simulink model "mars_rover_terrain"  (R2025a)
settings: Solver=daessc  StartTime=0.0  StopTime=130*10  FixedStep=1e-10  MaxStep=1e-1  RelTol=1e-3  AbsTol=1e-3  EnableMultiTasking=on
undefined symbols (not defined in the file): arm_q0, Control, eeConfig, L1, L2, L3, LS1, LS3, R1, R2, R3, Rover, rover_path, RS1, RS3, X, Y, Z
libraries: sm_lib x137, nesl_utility x109, fl_lib x85, sdl_lib x20, ee_lib x10, mars_rover_lib x8, simulink x4, slpidlib x3, batteryecm_lib x2, robotcorelib x1, robotalgslib x1
(part 1 of 10)
Description:
  | Mars Rover on Uneven Terrain
  | Copyright 2022-2025 The MathWorks, Inc.
settings Model: VariantFading=off  Creator=The MathWorks, Inc.  LastModifiedBy=smiller
settings SolverCC: AutoScaleAbsTol=off  MaxConsecutiveZCs=500  AlgebraicLoopSolver=TrustRegion  MinimalZcImpactIntegration=on
settings DataIOCC: MaxDataPoints=10000  SaveFormat=Array  ReturnWorkspaceOutputs=off  SignalLoggingName=logsout_mars_rover_terrain
settings OptimizationCC: ReuseModelBlockBuffer=off  LifeSpan=inf
settings DebuggingCC: UnconnectedInputMsg=warning  UnconnectedOutputMsg=warning  UnconnectedLineMsg=warning  AllowSymbolicDim=off  SFUnexpectedBacktrackingDiag=warning  SFNoUnconditionalDefaultTransitionDiag=warning  SFExecutionAtInitializationDiag=none  ArithmeticOperatorsInVariantConditions=warning
settings ModelReferenceCC: EnableRefExpFcnMdlSchedulingChecks=on
settings SFSimCC: SimUseLocalCustomCode=off  CustomCodeUndefinedFunction=UseInterfaceOnly
settings RTWCC: RTWUseLocalCustomCode=off  GPUComputeCapability=3.5  DLArmComputeVersion=19.05
settings CodeAppCC: StateflowObjectComments=on
settings GRTTargetCC: TargetLangStandard=C89/C90 (ANSI)
settings ConfigComp: CovMetricSettings=dw  CovSaveCumulativeToWorkspaceVar=on  CovSaveSingleToWorkspaceVar=on  CovExternalEMLEnable=off  CovSFcnEnable=off
settings SimscapeCC: SimscapeLogType=all  SimscapeLogSimulationStatistics=on  SimscapeLogName=simlog_mars_rover_terrain  SimscapeLogLimitData=off  SimscapeLogDataHistory=10000.0  SimscapeOperatingPoint=sm_mars_rover_op
settings DiagnosticsConfigSet: SimMechanicsConflictingReferenceFrames=none
settings ExplorerConfigSet: InternalSimMechanicsExplorerSettings="<ExplorerConfiguration><canonicalview>default</canonicalview><AnimationSetting><BasePlaybackSpeed>1.0</BasePlaybackSpeed><PlaybackSpeedFactor>16.0</PlaybackSpeedFactor></AnimationSetting><TilePanel><TileInfo><Tiles Columns=\"1\" Count=\"1\" Rows=\"1\"><Column Weight=\"1\"/><Row Weight=\"1\"/><Tile Height=\"1\" Width=\"1\" X=\"0\" Y=\"0\"/></Tiles></TileInfo><SceneInfo><SceneViewer><BGColor><R>0.819607853889465332</R><G>0.709803938865661621</G><B>0.662745118141174316</B></BGColor><Camera><DoPerspective>on</DoPerspective><Position><X>58.577415517520329</X><Y>32.9050911370938053</Y><Z>3.55732420536288174</Z></Position><Center><X>58.5375750727138282</X><Y>33.8739693483205073</Y><Z>3.31301343857646291</Z></Center><Up><X>0</X><Y>0</Y><Z>1</Z></Up><ViewLimDist>1</ViewLimDist><YLim>0.466307658154998583</YLim><XLim>1.07946358434775913</XLim></Camera></SceneViewer></SceneInfo></TilePanel><MechEditorPanel><Cameras><Camera><Id>Camera7</Id><Value><Name>Chassis_Rear</Name><NativeCamera><PositionTrackingFeature>Rover.Chassis.Chassis.Camera_Frames.Reference_Chassis_Camera_Rear.R</PositionTrackingFeature><CenterTrackingFeature>Rover.Chassis.Chassis.Camera_Frames.Reference_Chassis_Camera_Rear.R</CenterTrackingFeature><UpVectorTrackingFeature>Rover.World_Frame.W</UpVectorTrackingFeature><CenterTrackingOrigin>off</CenterTrackingOrigin><CenterTrackingDirection>-Y</CenterTrackingDirection><UpVectorTrackingDirection>+Z</UpVectorTrackingDirection></NativeCamera></Value></Camera><Camera><Id>Camera8</Id><Value><Name>Chassis_Right</Name><NativeCamera><PositionTrackingFeature>Rover.Chassis.Chassis.Camera_Frames.Reference_Chassis_Camera_Right.R</PositionTrackingFeature><CenterTrackingFeature>Rover.Chassis.Chassis.Camera_Frames.Reference_Chassis_Camera_Right.R</CenterTrackingFeature><UpVectorTrackingFeature>Rover.World_Frame.W</UpVectorTrackingFeature><CenterTrackingOrigin>off</CenterTrackingOrigin><CenterTrackingDirection>+X</CenterTrackingDirection><UpVectorTrackingDirection>+Z</UpVectorTrackingDirection></NativeCamera></Value></Camera><Camera><Id>Camera9</Id><Value><Name>Chassis_Top</Name><NativeCamera><PositionTrackingFeature>Rover.Chassis.Chassis.Camera_Frames.Reference_Chassis_Camera_Top.R</PositionTrackingFeature><CenterTrackingFeature>Rover.Chassis.Chassis.Camera_Frames.Reference_Chassis_Camera_Top.R</CenterTrackingFeature><UpVectorTrackingFeature>Rover.World_Frame.W</UpVectorTrackingFeature><CenterTrackingOrigin>off</CenterTrackingOrigin><CenterTrackingDirection>-Z</CenterTrackingDirection><UpVectorTrackingDirection>+Y</UpVectorTrackingDirection></NativeCamera></Value></Camera><Camera><Id>Camera10</Id><Value><Name>Whl_L1</Name><NativeCamera><PositionTrackingFeature>Rover.Chassis.Roll_and_Steer.Drive.Camera_Frame_L1.Reference_Cam_Whl.R</PositionTrackingFeature><CenterTrackingFeature>Rover.Chassis.Roll_and_Steer.Drive.Camera_Frame_L1.Reference_Cam_Whl.R</CenterTrackingFeature><UpVectorTrackingFeature>Rover.Chassis.Roll_and_Steer.Drive.Camera_Frame_L1.Reference_Cam_Whl.R</UpVectorTrackingFeature><CenterTrackingOrigin>off</CenterTrackingOrigin><CenterTrackingDirection>-Z</CenterTrackingDirection><UpVectorTrackingDirection>+X</UpVectorTrackingDirection></NativeCamera></Value></Camera><Camera><Id>Camera11</Id><Value><Name>Whl_R1</Name><NativeCamera><PositionTrackingFeature>Rover.Chassis.Roll_and_Steer.Drive.Camera_Frame_R1.Reference_Cam_Whl.R</PositionTrackingFeature><CenterTrackingFeature>Rover.Chassis.Roll_and_Steer.Drive.Camera_Frame_R1.Reference_Cam_Whl.R</CenterTrackingFeature><UpVectorTrackingFeature>Rover.Chassis.Roll_and_Steer.Drive.Camera_Frame_R1.Reference_Cam_Whl.R</UpVectorTrackingFeature><CenterTrackingOrigin>off</CenterTrackingOrigin><CenterTrackingDirection>+Z</CenterTrackingDirection><UpVectorTrackingDirection>-X</UpVectorTrackingDirection></NativeCamera></Value></Camera><Camera><Id>Camera12</Id><Value><Name>Whl_L2</Name><NativeCamera><PositionTrackingFeature>Rover.Chassis.Roll_and_Steer.Drive.Camera_Frame_L2.Reference_Cam_Whl.R</PositionTrackingFeature><CenterTrackingFeature>Rover.Chassis.Roll_and_Steer.Drive.Camera_Frame_L2.Reference_Cam_Whl.R</CenterTrackingFeature><UpVectorTrackingFeature>Rover.Chassis.Roll_and_Steer.Drive.Camera_Frame_L2.Reference_Cam_Whl.R</UpVectorTrackingFeature><CenterTrackingOrigin>off</CenterTrackingOrigin><CenterTrackingDirection>-Z</CenterTrackingDirection><UpVectorTrackingDirection>-Y</UpVectorTrackingDirection></NativeCamera></Value></Camera><Camera><Id>Camera13</Id><Value><Name>Whl_R2</Name><NativeCamera><PositionTrackingFeature>Rover.Chassis.Roll_and_Steer.Drive.Camera_Frame_R2.Reference_Cam_Whl.R</PositionTrackingFeature><CenterTrackingFeature>Rover.Chassis.Roll_and_Steer.Drive.Camera_Frame_R2.Reference_Cam_Whl.R</CenterTrackingFeature><UpVectorTrackingFeature>Rover.Chassis.Roll_and_Steer.Drive.Camera_Frame_R2.Reference_Cam_Whl.R</UpVectorTrackingFeature><CenterTrackingOrigin>off</CenterTrackingOrigin><CenterTrackingDirection>+Z</CenterTrackingDirection><UpVectorTrackingDirection>+Y</UpVectorTrackingDirection></NativeCamera></Value></Camera><Camera><Id>Camera14</Id><Value><Name>Whl_L3</Name><NativeCamera><PositionTrackingFeature>Rover.Chassis.Roll_and_Steer.Drive.Camera_Frame_L3.Reference_Cam_Whl.R</PositionTrackingFeature><CenterTrackingFeature>Rover.Chassis.Roll_and_Steer.Drive.Camera_Frame_L3.Reference_Cam_Whl.R</CenterTrackingFeature><UpVectorTrackingFeature>Rover.Chassis.Roll_and_Steer.Drive.Camera_Frame_L3.Reference_Cam_Whl.R</UpVectorTrackingFeature><CenterTrackingOrigin>off</CenterTrackingOrigin><CenterTrackingDirection>-Z</CenterTrackingDirection><UpVectorTrackingDirection>+X</UpVectorTrackingDirection></NativeCamera></Value></Camera><Camera><Id>Camera15</Id><Value><Name>Whl_R3</Name><NativeCamera><PositionTrackingFeature>Rover.Chassis.Roll_and_Steer.Drive.Camera_Frame_R3.Reference_Cam_Whl.R</PositionTrackingFeature><CenterTrackingFeature>Rover.Chassis.Roll_and_Steer.Drive.Camera_Frame_R3.Reference_Cam_Whl.R</CenterTrackingFeature><UpVectorTrackingFeature>Rover.Chassis.Roll_and_Steer.Drive.Camera_Frame_R3.Reference_Cam_Whl.R</UpVectorTrackingFeature><CenterTrackingOrigin>off</CenterTrackingOrigin><CenterTrackingDirection>+Z</CenterTrackingDirection><UpVectorTrackingDirection>-X</UpVectorTrackingDirection></NativeCamera></Value></Camera><Camera><Id>Camera16</Id><Value><Name>Chassis_FR</Name><NativeCamera><PositionTrackingFeature>Rover.Chassis.Chassis.Camera_Frames.Reference_Chassis_Camera_FR.R</PositionTrackingFeature><CenterTrackingFeature>Rover.Chassis.Chassis.Camera_Frames.Reference_Chassis_Camera_FR.R</CenterTrackingFeature><UpVectorTrackingFeature>Rover.World_Frame.W</UpVectorTrackingFeature><CenterTrackingOrigin>off</CenterTrackingOrigin><CenterTrackingDirection>+X</CenterTrackingDirection><UpVectorTrackingDirection>+Z</UpVectorTrackingDirection></NativeCamera></Value></Camera><Camera><Id>Camera17</Id><Value><Name>Chassis_Front</Name><NativeCamera><PositionTrackingFeature>Rover.Chassis.Chassis.Camera_Frames.Reference_Chassis_Camera_Front.R</PositionTrackingFeature><CenterTrackingFeature>Rover.Chassis.Chassis.Camera_Frames.Reference_Chassis_Camera_Front.R</CenterTrackingFeature><UpVectorTrackingFeature>Rover.World_Frame.W</UpVectorTrackingFeature><CenterTrackingOrigin>off</CenterTrackingOrigin><CenterTrackingDirection>+X</CenterTrackingDirection><UpVectorTrackingDirection>+Z</UpVectorTrackingDirection></NativeCamera></Value></Camera><Camera><Id>Camera18</Id><Value><Name>Chassis_WhlFR</Name><NativeCamera><PositionTrackingFeature>Rover.Chassis.Chassis.Camera_Frames.Reference_Chassis_Camera_WhlFR.R</PositionTrackingFeature><CenterTrackingFeature>Rover.Chassis.Chassis.Camera_Frames.Reference_Chassis_Camera_WhlFR.R</CenterTrackingFeature><UpVectorTrackingFeature>Rover.World_Frame.W</UpVectorTrackingFeature><CenterTrackingOrigin>off</CenterTrackingOrigin><CenterTrackingDirection>+X</CenterTrackingDirection><UpVectorTrackingDirection>+Z</UpVectorTrackingDirection></NativeCamera></Value></Camera><Camera><Id>Camera19</Id><Value><Name>Chassis_WhlRR</Name><NativeCamera><PositionTrackingFeature>Rover.Chassis.Chassis.Camera_Frames.Reference_Chassis_Camera_WhlRR.R</PositionTrackingFeature><CenterTrackingFeature>Rover.Chassis.Chassis.Camera_Frames.Reference_Chassis_Camera_WhlRR.R</CenterTrackingFeature><UpVectorTrackingFeature>Rover.World_Frame.W</UpVectorTrackingFeature><CenterTrackingOrigin>off</CenterTrackingOrigin><CenterTrackingDirection>+X</CenterTrackingDirection><UpVectorTrackingDirection>+Z</UpVectorTrackingDirection></NativeCamera></Value></Camera><Camera><Id>Camera20</Id><Value><Name>Chassis_Camera_Lens</Name><NativeCamera><PositionTrackingFeature>Rover.Chassis.Camera.rsm_head_1_RIGID.Reference_Camera.R</PositionTrackingFeature><CenterTrackingFeature>Rover.Chassis.Camera.rsm_head_1_RIGID.Reference_Camera.R</CenterTrackingFeature><UpVectorTrackingFeature>Rover.Chassis.Camera.rsm_head_1_RIGID.Reference_Camera.R</UpVectorTrackingFeature><CenterTrackingOrigin>off</CenterTrackingOrigin><CenterTrackingDirection>+Z</CenterTrackingDirection><UpVectorTrackingDirection>+X</UpVectorTrackingDirection></NativeCamera></Value></Camera></Cameras><GfxPanelCameraMap><MapElement CameraMLId=\"Camera8\" GfxPanelIndex=\"0\"/></GfxPanelCameraMap><VideoCreator><PlaybackSpeedRatio>1.0</PlaybackSpeedRatio><FrameRate>30</FrameRate><VideoFormat>MPEG-4</VideoFormat><FrameSize>auto</FrameSize></VideoCreator></MechEditorPanel></ExplorerConfiguration>"

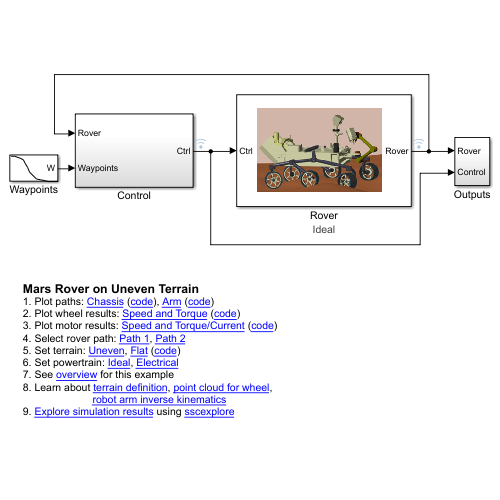
[thumbnail: Simulink's stored preview of the top-level diagram]
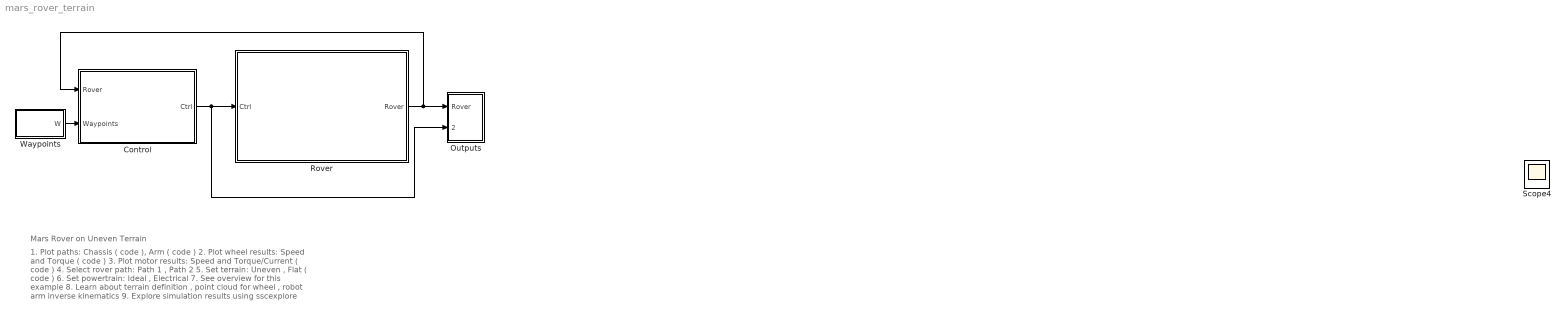
== system mars_rover_terrain ==
  note: Mars Rover on Uneven Terrain
  note: 1. Plot paths: Chassis ( code ), Arm ( code )
      | 2. Plot wheel results: Speed and Torque ( code )
      | 3. Plot motor results: Speed and Torque/Current ( code )
      | 4. Select rover path: Path 1 , Path 2
      | 5. Set terrain: Uneven , Flat ( code )
      | 6. Set powertrain: Ideal , Electrical
      | 7. See overview for this example
      | 8. Learn about terrain definition , point cloud for wheel ,
      | robot arm inverse kinematics
      | 9. Explore simulation results using sscexplore
  Control : Subsystem
  Outputs : Subsystem
  Rover : Subsystem
      mask init:
      | set_param(gcb,'AttributesFormatString',get_param([gcb '/Chassis/Powertrain'],'LabelModeActiveChoice'))
      settings: AttributesFormatString=Ideal
      mask Display: image('mars_rover_terrain_rover.png')
  Waypoints : Subsystem
      mask Display:
      | px = evalin('base','rover_path.x');
      | py = evalin('base','rover_path.y');
      | plot(px,py)
  Scope4 : Scope
      settings: ActiveDisplayYMinimum=-0.1776  ActiveDisplayYMaximum=0.10656  DataLoggingVariableName=ScopeData5
  wires:
  Waypoints/1(W) -> Control/2(Waypoints)
  Control/1(Ctrl) -> Outputs/2(Control), Rover/1(Ctrl)
  Rover/1(Rover) -> Control/1(Rover), Outputs/1(Rover)

== system mars_rover_terrain/Control ==
  In Bus Element : Inport  PortName=Rover  Element=Arm
  In Bus Element1 : Inport  PortName=Rover  Element=Chassis
  In Bus Element3 : Inport  PortName=Rover  Element=Sample
  In Bus Element5 : Inport  PortName=Rover  Element=Body
  Waypoints : Inport  Port=2
  Arm Control : Subsystem
  Chassis Control : Subsystem
  Out Bus Element : Outport  PortName=Ctrl  Element=Arm
  Out Bus Element1 : Outport  PortName=Ctrl  Element=Chassis
  wires:
  Chassis Control/1(RoverAtGoal) -> Arm Control/3(RoverAtGoal)
  Arm Control/1(Ctrl) -> Out Bus Element/1
  Waypoints/1 -> Chassis Control/1(Waypoints)
  Chassis Control/2(Ctrl) -> Out Bus Element1/1
  In Bus Element/1 -> Arm Control/1(Arm)
  In Bus Element1/1 -> Chassis Control/2(Chassis)
  In Bus Element3/1 -> Arm Control/2(Sensing)
  In Bus Element5/1 -> Chassis Control/3(Body)

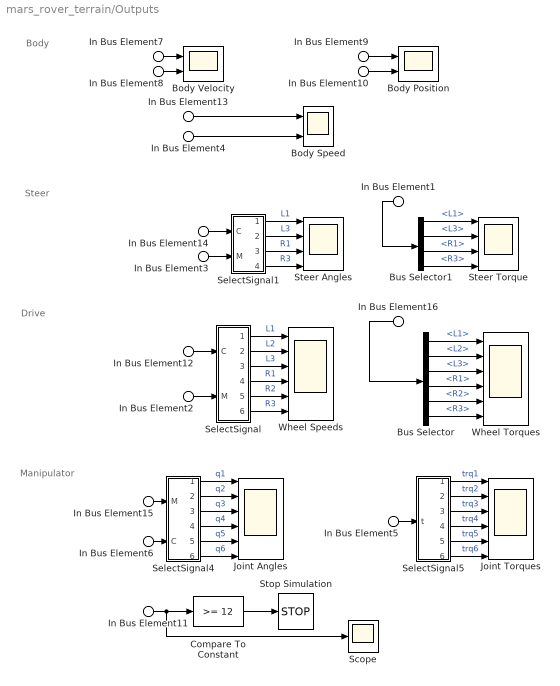
== system mars_rover_terrain/Outputs ==
  note: Body
  note: Steer
  note: Drive
  note: Manipulator
  In Bus Element2 : Inport  PortName=Rover  Element=Chassis.Wheels.Drive
  In Bus Element16 : Inport  PortName=Rover  Element=Chassis.Wheels.Drive.trq
  In Bus Element3 : Inport  PortName=Rover  Element=Chassis.Wheels.Steer
  In Bus Element15 : Inport  PortName=Rover  Element=Arm.q
  In Bus Element7 : Inport  PortName=Rover  Element=Body.vxy
  In Bus Element8 : Inport  PortName=Rover  Element=Body.wz
  In Bus Element9 : Inport  PortName=Rover  Element=Body.xyz
  In Bus Element10 : Inport  PortName=Rover  Element=Body.rpy
  In Bus Element4 : Inport  PortName=Rover  Element=Body.v
  In Bus Element1 : Inport  Port=2  PortName=Control  Element=Chassis.Steer
  In Bus Element12 : Inport  Port=2  PortName=Control  Element=Chassis.Cmd.wWhl
  In Bus Element13 : Inport  Port=2  PortName=Control  Element=Chassis.Cmd.v
  In Bus Element14 : Inport  Port=2  PortName=Control  Element=Chassis.Cmd.qSteer
  In Bus Element5 : Inport  Port=2  PortName=Control  Element=Arm.trq
  In Bus Element6 : Inport  Port=2  PortName=Control  Element=Arm.qCmd
  In Bus Element11 : Inport  Port=2  PortName=Control  Element=Arm.Mode
  Body Position : Scope  NumInputPorts=2
      settings: Title=Rover Position and Orientation  ActiveDisplayYMinimum=-4.54452  ActiveDisplayYMaximum=67.13718  YLabel=Rover XYZ Position (m)  DataLoggingVariableName=ScopeData2
  Body Speed : Scope  NumInputPorts=2
      settings: ActiveDisplayYMinimum=-0.0042  ActiveDisplayYMaximum=0.03782  DataLoggingVariableName=ScopeData7
  Body Velocity : Scope  NumInputPorts=2
      settings: Title=Rover Linear and Ang Velocities  ActiveDisplayYMinimum=-0.35082  ActiveDisplayYMaximum=0.38387  YLabel=Rover Linear Vel (m/s)
  Bus Selector : BusSelector  OutputSignals=L1,L2,L3,R1,R2,R3
  Bus Selector1 : BusSelector  OutputSignals=trq.L1,trq.L3,trq.R1,trq.R3
  Compare To Constant : simulink/Logic and Bit Operations/Compare To Constant  relop=>=  const=12  OutDataTypeStr=boolean
  Joint Angles : Scope  NumInputPorts=6
      settings: Title=Joint 1  ActiveDisplayYMinimum=-13.90292  ActiveDisplayYMaximum=99.39774  YLabel=Joint Angle (deg)  DataLoggingVariableName=ScopeData2
  Joint Torques : Scope  NumInputPorts=6
      settings: Title=Joint 1  ActiveDisplayYMinimum=-1231.55572  ActiveDisplayYMaximum=1377.74123  YLabel=Torque (N*m)
  Scope : Scope
      settings: ActiveDisplayYMinimum=-1.5  ActiveDisplayYMaximum=13.5
  SelectSignal : Subsystem
  SelectSignal1 : Subsystem
  SelectSignal4 : Subsystem
  SelectSignal5 : Subsystem
  Steer Angles : Scope  NumInputPorts=4
      settings: ActiveDisplayYMinimum=-23.51402  ActiveDisplayYMaximum=36.5986  YLabel=Steer Angle (Deg)  DataLoggingVariableName=ScopeData3
  Steer Torque : Scope  NumInputPorts=4
      settings: ActiveDisplayYMinimum=-139.38584  ActiveDisplayYMaximum=135.19843  YLabel=Torque (N*m)  DataLoggingVariableName=ScopeData4
  Stop Simulation : Stop
  Wheel Speeds : Scope  NumInputPorts=6
      settings: ActiveDisplayYMinimum=-0.5  ActiveDisplayYMaximum=4  YLabel=Wheel Speed (rad/s)  DataLoggingVariableName=ScopeData5
  Wheel Torques : Scope  NumInputPorts=6
      settings: ActiveDisplayYMinimum=17.86848  ActiveDisplayYMaximum=20.11099  YLabel=Torque (N*m)  DataLoggingVariableName=ScopeData6
  wires:
  In Bus Element4/1 -> Body Speed/2
  In Bus Element8/1 -> Body Velocity/2
  In Bus Element7/1 -> Body Velocity/1
  In Bus Element16/1 -> Bus Selector/1
  SelectSignal1/2(L3) -> Steer Angles/2  "L3"
  In Bus Element9/1 -> Body Position/1
  Bus Selector/3 -> Wheel Torques/3  "<L3>"
  In Bus Element10/1 -> Body Position/2
  Bus Selector/6 -> Wheel Torques/6  "<R3>"
  SelectSignal/3(L3) -> Wheel Speeds/3  "L3"
  SelectSignal/1(L1) -> Wheel Speeds/1  "L1"
  SelectSignal/6(R3) -> Wheel Speeds/6  "R3"
  Bus Selector/1 -> Wheel Torques/1  "<L1>"
  SelectSignal1/4(R3) -> Steer Angles/4  "R3"
  SelectSignal/2(L2) -> Wheel Speeds/2  "L2"
  SelectSignal/5(R2) -> Wheel Speeds/5  "R2"
  Bus Selector/2 -> Wheel Torques/2  "<L2>"
  SelectSignal/4(R1) -> Wheel Speeds/4  "R1"
  SelectSignal1/1(L1) -> Steer Angles/1  "L1"
  SelectSignal1/3(R1) -> Steer Angles/3  "R1"
  In Bus Element13/1 -> Body Speed/1
  Bus Selector/4 -> Wheel Torques/4  "<R1>"
  Bus Selector/5 -> Wheel Torques/5  "<R2>"
  In Bus Element1/1 -> Bus Selector1/1
  Bus Selector1/1 -> Steer Torque/1  "<L1>"
  Bus Selector1/2 -> Steer Torque/2  "<L3>"
  Bus Selector1/3 -> Steer Torque/3  "<R1>"
  Bus Selector1/4 -> Steer Torque/4  "<R3>"
  In Bus Element2/1 -> SelectSignal/2(M)
  In Bus Element3/1 -> SelectSignal1/2(M)
  In Bus Element5/1 -> SelectSignal5/1(t)
  SelectSignal4/1(q1) -> Joint Angles/1  "q1"
  In Bus Element15/1 -> SelectSignal4/1(M)
  SelectSignal5/1(t1) -> Joint Torques/1  "trq1"
  SelectSignal5/4(t4) -> Joint Torques/4  "trq4"
  SelectSignal4/4(q4) -> Joint Angles/4  "q4"
  SelectSignal4/2(q2) -> Joint Angles/2  "q2"
  SelectSignal5/5(t5) -> Joint Torques/5  "trq5"
  SelectSignal5/3(t3) -> Joint Torques/3  "trq3"
  SelectSignal5/2(t2) -> Joint Torques/2  "trq2"
  SelectSignal5/6(t6) -> Joint Torques/6  "trq6"
  SelectSignal4/3(q3) -> Joint Angles/3  "q3"
  SelectSignal4/6(q6) -> Joint Angles/6  "q6"
  SelectSignal4/5(q5) -> Joint Angles/5  "q5"
  In Bus Element6/1 -> SelectSignal4/2(C)
  In Bus Element12/1 -> SelectSignal/1(C)
  In Bus Element14/1 -> SelectSignal1/1(C)
  In Bus Element11/1 -> Scope/1, Compare To Constant/1
  Compare To Constant/1 -> Stop Simulation/1

== system mars_rover_terrain/Rover ==
  In Bus Element : Inport  PortName=Ctrl  Element=Arm.trq
  In Bus Element1 : Inport  PortName=Ctrl  Element=Arm.Sample
  In Bus Element3 : Inport  PortName=Ctrl  Element=Chassis
  Arm : mars_rover_lib/Arm  arm_q0_deg=arm_q0
  Chassis : Subsystem
      settings: PortSchema="{\"entries\":[{\"content\":{\"sides\":[{\"content\":{\"connectorIds\":[\"LConn1\",\"LConn2\",\"In1\",\"LConn3\",\"LConn4\"]},\"type\":\"ConnectorPlacement.EquallySpacedRectSide\",\"uuid\":\"1e8a3e2b-b3ca-4467-863a-9c237d71771f\"},{\"content\":{\"connectorIds\":[\"Out1\"],\"side\":\"RIGHT\"},\"type\":\"ConnectorPlacement.EquallySpacedRectSide\",\"uuid\":\"1c304fdb-ff64-4dc8-bd28-208b239a200a\"},{\"content\":{\"connectorIds\":[],\"side\":\"TOP\"},\"type\":\"ConnectorPlacement.EquallySpacedRectSide\",\"uuid\":\"6fd19973-5814-4525-bce6-20dd9c942e44\"}]},\"type\":\"ConnectorPlacement.EquallySpacedConnector\",\"uuid\":\"720db96a-3f3b-4ddd-a986-ea75ab459e47\"}],\"packageUris\":[\"http://schema.mathworks.com/mf0/Connector/R2020b\"],\"version\":\"1.0\"}"
      mask Display: image('mars_rover_terrain_chassis.png');
  Chassis DOF : Subsystem  mask{x0=rover_path.x(1), y0=rover_path.y(1), z0=rover_path.t0.pzOffset, yaw0=rover_path.t0.yaw, pitch_0=rover_path.t0.pitch, roll_0=rover_path.t0.roll}
      mask prompts: x0 "Chassis Initial Position x (m)"; y0 "Chassis Initial Position y (m)"; z0 "Chassis Initial Position z (m)"; yaw0 "Chassis Initial Orientation Yaw (rad)"; pitch_0 "Chassis Initial Orientation Pitch (rad)"; roll_0 "Chassis Initial Orientation Roll (rad)"
  Mechanism Configuration : sm_lib/Utilities/Mechanism Configuration  UniformGravity=Constant  GravityVector=[0 0 -3.72076]  GravityVectorUnits=m/s^2  LinearizationDelta=0.001  JointModeTransitionNonlinearIterations=2
  Path : Subsystem
      mask Display: image('mars_rover_terrain_path.png');
  Sample : Subsystem
      mask Display: image('mars_rover_terrain_sample.png');
  Solver Configuration : nesl_utility/Solver Configuration  PhysicalDomain=network_engine_domain  SubClassName=solver  LeftPortType=input  RightPortType=generic  Tones=[]  Harmonics=[]  SimulateNoise=off  Profile=off  UseLocalSampling=off  EnableSwitchedLinearOptims=on  FrequencyDomain=off  UseCCode=off  RelTol=0.001  AbsTol=1e-06  MinStep=1e-09  ToWorkspace=off  RevertToSquareIcSolve=off  NumHomotopyIterations=100  PhasorMode=off  PhasorModeNumHarmonics=1  ConsistencySolver=NEWTON_FTOL  IndexReductionMethod=DerivativeReplacement  DoDC=off  ResidualTolerance=1e-09  ConsistencyTolSource=GLOBAL  ConsistencyAbsTol=0.001  ConsistencyRelTol=0.001  ConsistencyTolFactor=0.001  UseLocalSolver=off  LocalSolverChoice=NE_BACKWARD_EULER_ADVANCER  ResolveIndetEquations=on  FunctionEvalNumThread=1  LocalSolverSampleTime=0.001  DoFixedCost=off  MaxNonlinIter=3  MaxModeIter=2  ComputeImpulses=off  ImpulseIterations=2  LinearAlgebra=auto  LinearAlgebraNumThread=0  EquationFormulation=NE_TIME_EF  DelaysMemoryBudget=1024  AutomaticFiltering=on  FilteringTimeConstant=0.001  PartitionStorageMethod=AS_NEEDED  PartitionMemoryBudget=1024  PartitionMethod=FAST  MultibodyUseLocalSolver=off  MultibodyLocalSolverChoice=ODE1  MultibodyLocalSolverSampleTime=0.001
  Terrain : Subsystem
      mask Display: image('mars_rover_terrain_terrain.png');
  World Frame : sm_lib/Frames and Transforms/World Frame
  Out Bus Element : Outport  PortName=Rover  Element=Arm
  Out Bus Element1 : Outport  PortName=Rover  Element=Chassis
  Out Bus Element3 : Outport  PortName=Rover  Element=Sample
  Out Bus Element4 : Outport  PortName=Rover  Element=Body
  wires:
  In Bus Element/1 -> Arm/1
  In Bus Element1/1 -> Sample/1(Ctrl)
  In Bus Element3/1 -> Chassis/1(Ctrl)
  Arm/1 -> Out Bus Element/1
  Sample/1(m) -> Out Bus Element3/1
  Chassis DOF/1(m) -> Out Bus Element4/1
  Chassis/1(m) -> Out Bus Element1/1
  connections:
  Chassis/LConn1 -- Arm/LConn2 -- Sample/RConn2
  Terrain/RConn2 -- Chassis/LConn4
  Chassis DOF/RConn1 -- Chassis/LConn3
  Arm/LConn1 -- Sample/RConn1
  Sample/RConn3 -- Chassis/LConn2
  Terrain/RConn1 -- Sample/LConn1 -- Mechanism Configuration/RConn1 -- Solver Configuration/RConn1 -- Path/LConn1 -- Chassis DOF/LConn1 -- World Frame/RConn1

== system mars_rover_terrain/Waypoints ==
  Matrix Concatenate : Concatenate  Mode=Multidimensional array  ConcatenateDimension=2
  rover path x : Constant  Value=rover_path.x
  rover path y : Constant  Value=rover_path.y
  W : Outport
  wires:
  rover path x/1 -> Matrix Concatenate/1
  rover path y/1 -> Matrix Concatenate/2
  Matrix Concatenate/1 -> W/1

== system mars_rover_terrain/Control/Arm Control ==
  In Bus Element1 : Inport  PortName=Arm
  In Bus Element2 : Inport  Port=2  PortName=Sensing
  RoverAtGoal : Inport  Port=3
  " Trajectory Planner" : Subsystem
  Add : Sum  Inputs=+-
  Bus Creator : BusCreator  Inputs=3
  Bus to Vec q : Subsystem
  PID Control : slpidlib/PID Controller  Controller=PID  Form=Parallel  TimeDomain=Continuous-time  UseExternalTs=off  SampleTime=-1  IntegratorMethod=Forward Euler  FilterMethod=Forward Euler  ControllerParametersSource=internal  P=Control.Arm.Kp  I=Control.Arm.Ki  UseKiTs=off  D=Control.Arm.Kd  UseExternalDerivativeSource=off  N=Control.Arm.N  UseFilter=on  TunerSelectOption=Transfer Function Based (PID Tuner App)  InitialConditionSource=internal  InitialConditionForIntegrator=0  InitialConditionForFilter=0  DifferentiatorICPrevScaledInput=0  ExternalReset=none  TrackingMode=off  Kt=1  LimitOutput=off  SatLimitsSource=internal  UpperSaturationLimit=inf  LowerSaturationLimit=-inf  LinearizeAsGain=on  AntiWindupMode=none  Kb=1  LimitIntegrator=off  UpperIntegratorSaturationLimit=inf  LowerIntegratorSaturationLimit=-inf  POutMin=[]  POutMax=[]  IOutMin=[]  IOutMax=[]  DOutMin=[]  DOutMax=[]  NOutMin=[]  NOutMax=[]  SumOutMin=[]  SumOutMax=[]  SaturationOutMin=[]  SaturationOutMax=[]  PParamMin=[]  PParamMax=[]  IParamMin=[]  IParamMax=[]  DParamMin=[]  DParamMax=[]  NParamMin=[]  NParamMax=[]  KbParamMin=[]  KbParamMax=[]  KtParamMin=[]  KtParamMax=[]  KbOutMin=[]  KbOutMax=[]  KtOutMin=[]  KtOutMax=[]  IntegratorOutMin=[]  IntegratorOutMax=[]  FilterOutMin=[]  FilterOutMax=[]  SumI1OutMin=[]  SumI1OutMax=[]  SumI2OutMin=[]  SumI2OutMax=[]  SumI3OutMin=[]  SumI3OutMax=[]  SumI4OutMin=[]  SumI4OutMax=[]  SumDOutMin=[]  SumDOutMax=[]  DifferentiatorOutMin=[]  DifferentiatorOutMax=[]  FilterDiffOutCoefMin=[]  FilterDiffOutCoefMax=[]  ReciprocalOutMin=[]  ReciprocalOutMax=[]  SumDenOutMin=[]  SumDenOutMax=[]  SumNumOutMin=[]  SumNumOutMax=[]  DivideOutMin=[]  DivideOutMax=[]  UdiffTsProdOutMin=[]  UdiffTsProdOutMax=[]  NTsProdOutMin=[]  NTsProdOutMax=[]  UintegralTsProdOutMin=[]  UintegralTsProdOutMax=[]  UngainTsProdOutMin=[]  UngainTsProdOutMax=[]  ClampingZeroOutDataTypeStr=Inherit: Inherit via back propagation  ClampingZeroOutMin=[]  ClampingZeroOutMax=[]  FilterDenConstantOutDataTypeStr=Inherit: Inherit via back propagation  FilterDenConstantOutMin=[]  FilterDenConstantOutMax=[]  PCopyOutDataTypeStr=Inherit: Inherit via back propagation  PCopyOutMin=[]  PCopyOutMax=[]  NCopyOutDataTypeStr=Inherit: Inherit via back propagation  NCopyOutMin=[]  NCopyOutMax=[]  IntegratorContinuousStateAttributes=''  IntegratorStateMustResolveToSignalObject=off  IntegratorRTWStateStorageClass=Auto  FilterContinuousStateAttributes=''  FilterStateMustResolveToSignalObject=off  FilterRTWStateStorageClass=Auto  ParallelPVariant=InternalParameters  IdealPVariant=Disabled  IVariant=InternalParameters  DVariant=InternalParameters  IntegratorVariant=Continuous  SatVariant=Disabled  AWVariant=Passthrough  PCopyVariant=Disabled  TRVariant=Disabled  FdbkBlocksVariant=Forward  IdealPFdbkVariant=Disabled  SatFdbkVariant=Disabled  DerivativeFilterVariant=ContFilter  NVariant=InternalParameters  NCopyVariant=Disabled  FilterICVariant=InternalICsFilter  IntegratorICVariant=InternalICs  ExternalResetVariant=Disabled  TRSumVariant=Passthrough  SumFdbkVariant=Disabled  SumVariant=Sum_PID  TsampFilterVariant=InternalTs  TsampNgainVariant=Passthrough  TsampIntegralVariant=Disabled_SignalSpec  ExternalSaturationOutDataTypeStr=Inherit: Same as second input  DerivativeSourceVariant=ErrorSignal  PreIntVariant=InternalPreInt
  Vec to Bus q : Subsystem
  Vec to Bus trq : Subsystem
  Bus Element Out : Outport  PortName=Ctrl  Element=trq
  Out Bus Element : Outport  PortName=Ctrl  Element=Sample
  Out Bus Element1 : Outport  PortName=Ctrl  Element=qCmd
  Bus Element Out1 : Outport  PortName=Ctrl  Element=Mode
  wires:
  " Trajectory Planner"/5(Cmd Angles) -> Vec to Bus q/1(V), Add/1
  PID Control/1 -> Vec to Bus trq/1(V)
  Bus to Vec q/1(V) -> Add/2, " Trajectory Planner"/3(Arm Angles)
  Add/1 -> PID Control/1
  RoverAtGoal/1 -> " Trajectory Planner"/1(RoverAtGoal)
  " Trajectory Planner"/1(Hold) -> Bus Creator/1  "Hold"
  " Trajectory Planner"/2(Stored) -> Bus Creator/2  "Stored"
  Vec to Bus trq/1(B) -> Bus Element Out/1
  Bus Creator/1 -> Out Bus Element/1
  Vec to Bus q/1(B) -> Out Bus Element1/1
  In Bus Element2/1 -> " Trajectory Planner"/2(Sensing)
  In Bus Element1/1 -> Bus to Vec q/1(B)
  " Trajectory Planner"/4(Mode) -> Bus Element Out1/1
  " Trajectory Planner"/3(Location) -> Bus Creator/3  "Location"

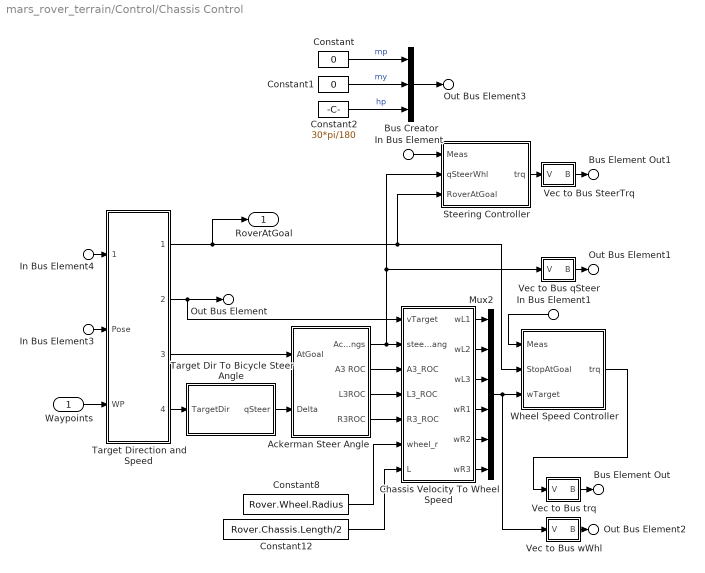
== system mars_rover_terrain/Control/Chassis Control ==
  Waypoints : Inport
  In Bus Element1 : Inport  Port=2  PortName=Chassis  Element=Wheels.Drive
  In Bus Element : Inport  Port=2  PortName=Chassis  Element=Wheels.Steer
  In Bus Element3 : Inport  Port=3  PortName=Body  Element=Pose
  In Bus Element4 : Inport  Port=3  PortName=Body  Element=v
  Ackerman Steer Angle : Subsystem
  Bus Creator : BusCreator  Inputs=3
  Chassis Velocity To Wheel Speed : MATLAB Function  TreatAsAtomicUnit=on
  Constant : Constant  Value=0
  Constant1 : Constant  Value=0
  Constant12 : Constant  Value=Rover.Chassis.Length/2
  Constant2 : Constant  Value=30*pi/180
  Constant8 : Constant  Value=Rover.Wheel.Radius
  Mux2 : Mux  Inputs=6
  Steering Controller : Subsystem  mask{Kp=Control.Steer.Kp, Ki=Control.Steer.Ki, Kd=Control.Steer.Kd, N=Control.Steer.N, Ts_Targetq=Control.Steer.FiltTargetq, Ts_Measq=Control.Steer.FiltSensorq, trq_max_pos=Control.Steer.TrqCmdLimitPos, trq_max_neg=Control.Steer.TrqCmdLimitNeg}
      mask prompts: Kp "Propotional Gain"; Ki "Integral Gain"; Kd "Derivative Gain"; N "Filter Constant (derivative)"; Ts_Targetq "Target Angle (deg)"; Ts_Measq "Sensed Angle (deg)"; trq_max_pos "Torque Command Upper Limit (N*m)"; trq_max_neg "Torque Command Lower Limit (N*m)"
      mask DialogControl cont_pid Prompt: PID Controller
      mask DialogControl cont_filt_ts Prompt: Filter Time Constants
      mask DialogControl cont_trqCmdLim Prompt: Limits at Wheel
  Target Dir To Bicycle Steer Angle : Subsystem  mask{L=1, ld=0.75}
      mask prompts: L "Bicycle length"; ld "Lookahead distance"
      mask TypeOptions L: Bicycle length/Value
      mask TypeOptions ld: Lookahead distance/Value
  Target Direction and Speed : Subsystem
  Vec to Bus SteerTrq : Subsystem
  Vec to Bus qSteer : Subsystem
  Vec to Bus trq : Subsystem
  Vec to Bus wWhl : Subsystem
  Wheel Speed Controller : Subsystem  mask{Kp=Control.Drive.Kp, Ki=Control.Drive.Ki, Kd=Control.Drive.Kd, N=Control.Drive.N, Ts_Targetw=Control.Drive.FiltTargetw, Ts_Measw=Control.Drive.FiltSensorw, trq_max_pos=Control.Drive.TrqCmdLimitPos, trq_max_neg=Control.Drive.TrqCmdLimitNeg}
      mask prompts: Kp "Propotional Gain"; Ki "Integral Gain"; Kd "Derivative Gain"; N "Filter Constant (derivative)"; Ts_Targetw "Target Speed (sec)"; Ts_Measw "Sensed Speed (sec)"; trq_max_pos "Torque Command Upper Limit (N*m)"; trq_max_neg "Torque Command Lower Limit (N*m)"
      mask DialogControl Container4 Prompt: PID Controller
      mask DialogControl cont_filt_ts Prompt: Filter Time Constants
      mask DialogControl cont_trqCmdLim Prompt: Limits
  RoverAtGoal : Outport
  Bus Element Out1 : Outport  Port=2  PortName=Ctrl  Element=Steer.trq
  Bus Element Out : Outport  Port=2  PortName=Ctrl  Element=Drive.trq
  Out Bus Element : Outport  Port=2  PortName=Ctrl  Element=Cmd.v
  Out Bus Element1 : Outport  Port=2  PortName=Ctrl  Element=Cmd.qSteer
  Out Bus Element2 : Outport  Port=2  PortName=Ctrl  Element=Cmd.wWhl
  Out Bus Element3 : Outport  Port=2  PortName=Ctrl  Element=Camera
  wires:
  Chassis Velocity To Wheel Speed/6(wR3) -> Mux2/6
  Mux2/1 -> Wheel Speed Controller/3(wTarget), Vec to Bus wWhl/1(V)
  Ackerman Steer Angle/4(R3ROC) -> Chassis Velocity To Wheel Speed/5(R3_ROC)
  Chassis Velocity To Wheel Speed/5(wR2) -> Mux2/5
  Chassis Velocity To Wheel Speed/4(wR1) -> Mux2/4
  Ackerman Steer Angle/1(AckSteerAngs) -> Steering Controller/2(qSteerWhl), Vec to Bus qSteer/1(V), Chassis Velocity To Wheel Speed/2(steer_ang)
  Chassis Velocity To Wheel Speed/3(wL3) -> Mux2/3
  Constant12/1 -> Chassis Velocity To Wheel Speed/7(L)
  Constant8/1 -> Chassis Velocity To Wheel Speed/6(wheel_r)
  Chassis Velocity To Wheel Speed/2(wL2) -> Mux2/2
  Chassis Velocity To Wheel Speed/1(wL1) -> Mux2/1
  Ackerman Steer Angle/3(L3ROC) -> Chassis Velocity To Wheel Speed/4(L3_ROC)
  Ackerman Steer Angle/2(A3 ROC) -> Chassis Velocity To Wheel Speed/3(A3_ROC)
  Target Dir To Bicycle Steer Angle/1(qSteer) -> Ackerman Steer Angle/2(Delta)
  Wheel Speed Controller/1(trq) -> Vec to Bus trq/1(V)
  Steering Controller/1(trq) -> Vec to Bus SteerTrq/1(V)
  Vec to Bus trq/1(B) -> Bus Element Out/1
  Vec to Bus SteerTrq/1(B) -> Bus Element Out1/1
  In Bus Element1/1 -> Wheel Speed Controller/1(Meas)
  In Bus Element/1 -> Steering Controller/1(Meas)
  Vec to Bus qSteer/1(B) -> Out Bus Element1/1
  Vec to Bus wWhl/1(B) -> Out Bus Element2/1
  Target Direction and Speed/1(StopAtGoal) -> Wheel Speed Controller/2(StopAtGoal), Steering Controller/3(RoverAtGoal), RoverAtGoal/1
  Target Direction and Speed/2(vTarget) -> Chassis Velocity To Wheel Speed/1(vTarget), Out Bus Element/1
  In Bus Element3/1 -> Target Direction and Speed/2(Pose)
  Waypoints/1 -> Target Direction and Speed/3(WP)
  Target Direction and Speed/3(AtGoal) -> Ackerman Steer Angle/1(AtGoal)
  Target Direction and Speed/4(TargetDir) -> Target Dir To Bicycle Steer Angle/1(TargetDir)
  In Bus Element4/1 -> Target Direction and Speed/1(vRover)
  Constant/1 -> Bus Creator/1  "mp"
  Constant1/1 -> Bus Creator/2  "my"
  Constant2/1 -> Bus Creator/3  "hp"
  Bus Creator/1 -> Out Bus Element3/1

== system mars_rover_terrain/Outputs/SelectSignal ==
  In Bus Element1 : Inport  PortName=C  Element=L1
  In Bus Element2 : Inport  PortName=C  Element=L2
  In Bus Element3 : Inport  PortName=C  Element=L3
  In Bus Element4 : Inport  PortName=C  Element=R1
  In Bus Element5 : Inport  PortName=C  Element=R2
  In Bus Element : Inport  PortName=C  Element=R3
  In Bus Element7 : Inport  Port=2  PortName=M  Element=w.L1
  In Bus Element10 : Inport  Port=2  PortName=M  Element=w.L2
  In Bus Element8 : Inport  Port=2  PortName=M  Element=w.L3
  In Bus Element11 : Inport  Port=2  PortName=M  Element=w.R3
  In Bus Element12 : Inport  Port=2  PortName=M  Element=w.R2
  In Bus Element9 : Inport  Port=2  PortName=M  Element=w.R1
  Mux{,1..5} (6 alike) : Mux  Inputs=2
  L1 : Outport
  L2 : Outport  Port=2
  L3 : Outport  Port=3
  R1 : Outport  Port=4
  R2 : Outport  Port=5
  R3 : Outport  Port=6
  wires:
  In Bus Element7/1 -> Mux/2  "Meas"
  Mux/1 -> L1/1
  In Bus Element1/1 -> Mux/1  "Cmd"
  In Bus Element2/1 -> Mux1/1  "Cmd"
  Mux1/1 -> L2/1
  In Bus Element10/1 -> Mux1/2  "Meas"
  In Bus Element8/1 -> Mux2/2  "Meas"
  Mux2/1 -> L3/1
  In Bus Element3/1 -> Mux2/1  "Cmd"
  In Bus Element4/1 -> Mux3/1  "Cmd"
  Mux3/1 -> R1/1
  In Bus Element9/1 -> Mux3/2  "Meas"
  In Bus Element12/1 -> Mux4/2  "Meas"
  Mux4/1 -> R2/1
  In Bus Element5/1 -> Mux4/1  "Cmd"
  In Bus Element/1 -> Mux5/1  "Cmd"
  Mux5/1 -> R3/1
  In Bus Element11/1 -> Mux5/2  "Meas"

== system mars_rover_terrain/Outputs/SelectSignal1 ==
  In Bus Element1 : Inport  PortName=C  Element=L1
  In Bus Element3 : Inport  PortName=C  Element=L3
  In Bus Element4 : Inport  PortName=C  Element=R3
  In Bus Element2 : Inport  PortName=C  Element=R1
  In Bus Element5 : Inport  Port=2  PortName=M  Element=q.L1
  In Bus Element6 : Inport  Port=2  PortName=M  Element=q.L3
  In Bus Element7 : Inport  Port=2  PortName=M  Element=q.R1
  In Bus Element8 : Inport  Port=2  PortName=M  Element=q.R3
  Mux{,1..3} (4 alike) : Mux  Inputs=2
  L1 : Outport
  L3 : Outport  Port=2
  R1 : Outport  Port=3
  R3 : Outport  Port=4
  wires:
  In Bus Element8/1 -> Mux3/2  "Meas"
  Mux3/1 -> R3/1
  In Bus Element2/1 -> Mux2/1  "Cmd"
  In Bus Element4/1 -> Mux3/1  "Cmd"
  Mux2/1 -> R1/1
  In Bus Element7/1 -> Mux2/2  "Meas"
  In Bus Element6/1 -> Mux1/2  "Meas"
  Mux1/1 -> L3/1
  In Bus Element1/1 -> Mux/1  "Cmd"
  In Bus Element3/1 -> Mux1/1  "Cmd"
  Mux/1 -> L1/1
  In Bus Element5/1 -> Mux/2  "Meas"

== system mars_rover_terrain/Outputs/SelectSignal4 ==
  In Bus Element1 : Inport  PortName=M  Element=q1
  In Bus Element2 : Inport  PortName=M  Element=q2
  In Bus Element3 : Inport  PortName=M  Element=q3
  In Bus Element4 : Inport  PortName=M  Element=q4
  In Bus Element5 : Inport  PortName=M  Element=q5
  In Bus Element6 : Inport  PortName=M  Element=q6
  In Bus Element7 : Inport  Port=2  PortName=C  Element=q1
  In Bus Element8 : Inport  Port=2  PortName=C  Element=q2
  In Bus Element9 : Inport  Port=2  PortName=C  Element=q3
  In Bus Element10 : Inport  Port=2  PortName=C  Element=q4
  In Bus Element11 : Inport  Port=2  PortName=C  Element=q5
  In Bus Element12 : Inport  Port=2  PortName=C  Element=q6
  Mux{,1..5} (6 alike) : Mux  Inputs=2
  q1 : Outport
  q2 : Outport  Port=2
  q3 : Outport  Port=3
  q4 : Outport  Port=4
  q5 : Outport  Port=5
  q6 : Outport  Port=6
  wires:
  In Bus Element6/1 -> Mux5/2  "Meas"
  Mux5/1 -> q6/1
  In Bus Element12/1 -> Mux5/1  "Cmd"
  In Bus Element11/1 -> Mux4/1  "Cmd"
  Mux4/1 -> q5/1
  In Bus Element5/1 -> Mux4/2  "Meas"
  In Bus Element4/1 -> Mux3/2  "Meas"
  Mux3/1 -> q4/1
  In Bus Element10/1 -> Mux3/1  "Cmd"
  In Bus Element9/1 -> Mux2/1  "Cmd"
  Mux2/1 -> q3/1
  Mux1/1 -> q2/1
  In Bus Element8/1 -> Mux1/1  "Cmd"
  In Bus Element7/1 -> Mux/1  "Cmd"
  Mux/1 -> q1/1
  In Bus Element1/1 -> Mux/2  "Meas"
  In Bus Element2/1 -> Mux1/2  "Meas"
  In Bus Element3/1 -> Mux2/2  "Meas"

== system mars_rover_terrain/Outputs/SelectSignal5 ==
  t : Inport
  Bus Selector : BusSelector  OutputSignals=t1,t2,t3,t4,t5,t6
  t1 : Outport
  t2 : Outport  Port=2
  t3 : Outport  Port=3
  t4 : Outport  Port=4
  t5 : Outport  Port=5
  t6 : Outport  Port=6
  wires:
  Bus Selector/1 -> t1/1  "<t1>"
  Bus Selector/2 -> t2/1  "<t2>"
  Bus Selector/3 -> t3/1  "<t3>"
  Bus Selector/4 -> t4/1  "<t4>"
  Bus Selector/5 -> t5/1  "<t5>"
  Bus Selector/6 -> t6/1  "<t6>"
  t/1 -> Bus Selector/1
